simulink model "boost_simulink"  (R2024a)
settings: Solver=VariableStepAuto  StartTime=0.0  StopTime=inf  FixedStep=0.01  RelTol=1e-3
StopFcn:
  | boostIO('close'); clear boostIO
libraries: simulink x1
settings Model: Creator=Razowan  LastModifiedBy=Razowan

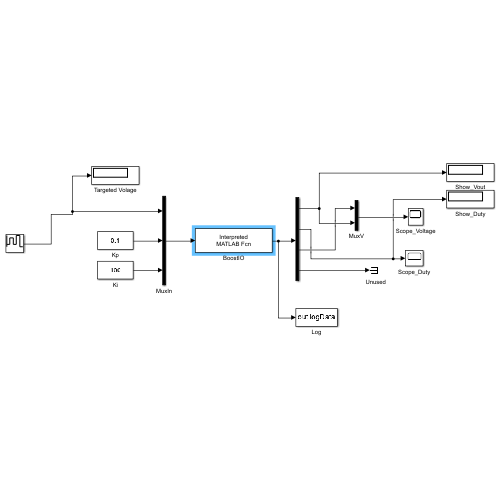
[thumbnail: Simulink's stored preview of the top-level diagram]
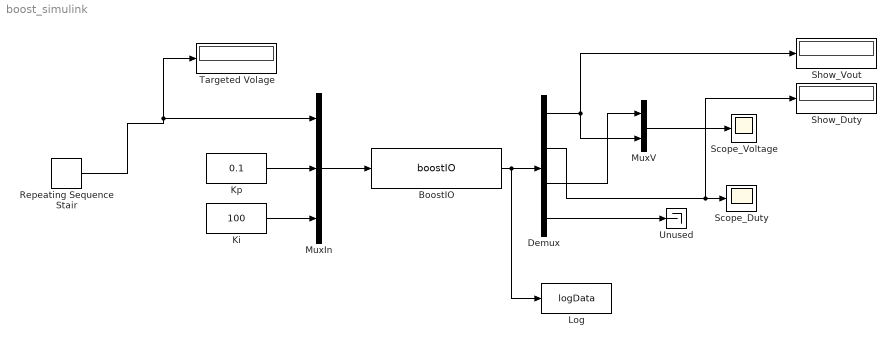
== system boost_simulink ==
  BoostIO : MATLABFcn  MATLABFcn=boostIO  OutputDimensions=4  OutputSignalType=real  SampleTime=0.01
  Demux : Demux
  Ki : Constant  Value=100
  Kp : Constant  Value=0.1
  Log : ToWorkspace  VariableName=logData  SampleTime=-1
  MuxIn : Mux  Inputs=3
  MuxV : Mux  Inputs=2
  Repeating Sequence Stair : simulink/Sources/Repeating Sequence Stair  OutValues=[10 15 10 17 8].'  tsamp=5  OutMin=[]  OutMax=[]  OutDataTypeStr=double  OutputDataTypeScalingMode=double  OutDataType=fixdt(0,8)  ConRadixGroup=Best Precision: Vector-wise  OutScaling=2^-12
  Scope_Duty : Scope
  Scope_Voltage : Scope
  Show_Duty : Display
  Show_Vout : Display
  Targeted Volage : Display
  Unused : Terminator
  wires:
  Repeating Sequence Stair/1 -> Targeted Volage/1, MuxIn/1
  Kp/1 -> MuxIn/2
  Ki/1 -> MuxIn/3
  MuxIn/1 -> BoostIO/1
  BoostIO/1 -> Log/1, Demux/1
  Demux/3 -> MuxV/1
  Demux/1 -> Show_Vout/1, MuxV/2
  MuxV/1 -> Scope_Voltage/1
  Demux/2 -> Scope_Duty/1, Show_Duty/1
  Demux/4 -> Unused/1
